simulink subsystem "Actuators"  (R2024b)
settings: Solver=VariableStepAuto  StartTime=0.0  StopTime=10.0  RelTol=1e-3
undefined symbols (not defined in the file): actuators, simulation
settings Model: Creator=marco  LastModifiedBy=domac

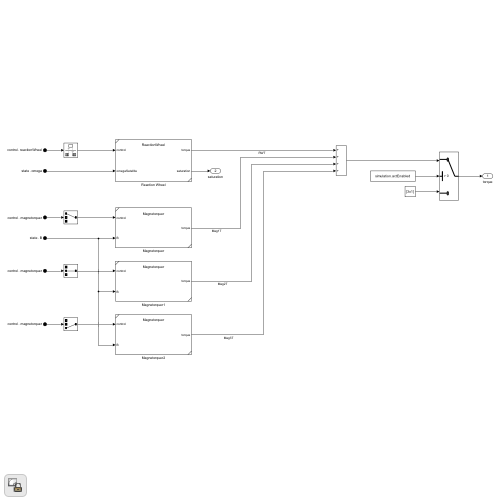
[thumbnail: Simulink's stored preview of the top-level diagram]
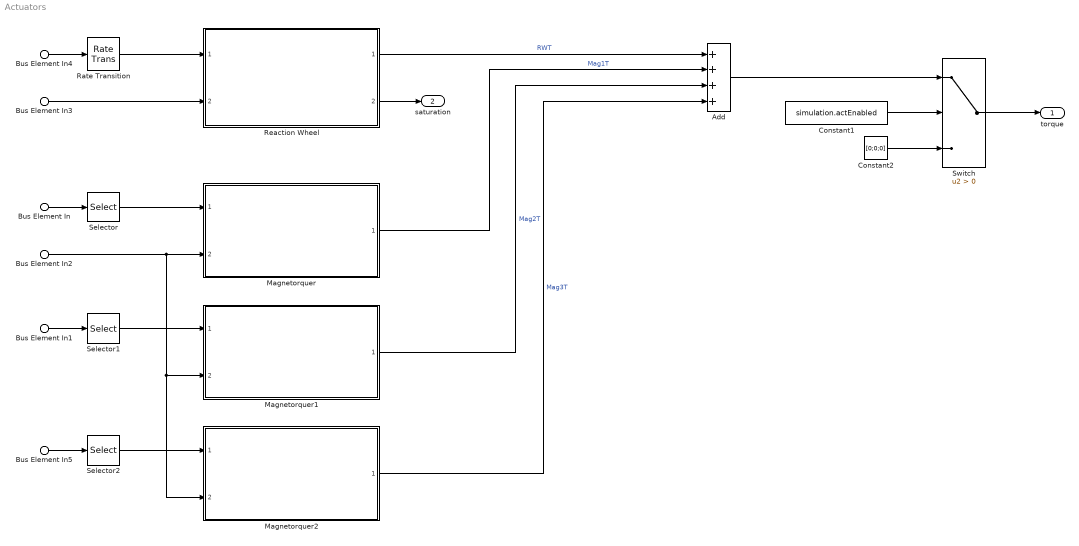
== system Actuators ==
  Bus Element In : Inport  PortName=control  Element=magnetorquer
  Bus Element In1 : Inport  PortName=control  Element=magnetorquer
  Bus Element In5 : Inport  PortName=control  Element=magnetorquer
  Bus Element In4 : Inport  PortName=control  Element=reactionWheel
  Bus Element In2 : Inport  Port=2  PortName=state  Element=B
  Bus Element In3 : Inport  Port=2  PortName=state  Element=omega
  Add : Sum  Inputs=++++
  Constant1 : Constant  Value=simulation.actEnabled
  Constant2 : Constant  Value=[0;0;0]  VectorParams1D=off
  Magnetorquer : Subsystem  ReferencedSubsystem=Magnetorquer  R=actuators.magnetorquer(1).R  k=actuators.magnetorquer(1).k
  Magnetorquer1 : Subsystem  ReferencedSubsystem=Magnetorquer  R=actuators.magnetorquer(2).R  k=actuators.magnetorquer(2).k
  Magnetorquer2 : Subsystem  ReferencedSubsystem=Magnetorquer  R=actuators.magnetorquer(3).R  k=actuators.magnetorquer(3).k
  Rate Transition : RateTransition  OutPortSampleTime=actuators.wheel.sTControl
  Reaction Wheel : Subsystem  ReferencedSubsystem=ReactionWheel  k=actuators.wheel.k  maxSpeed=actuators.wheel.maxSpeed  capacity=actuators.wheel.capacity  imbalance=actuators.wheel.imbalance  R=actuators.wheel.R  seed=0  torqueVariance=actuators.wheel.torqueVariance
  Selector : Selector  InputPortWidth=3  IndexOptions=Index vector (dialog)  Indices=1  OutputSizes=1
  Selector1 : Selector  InputPortWidth=3  IndexOptions=Index vector (dialog)  Indices=2  OutputSizes=1
  Selector2 : Selector  InputPortWidth=3  IndexOptions=Index vector (dialog)  Indices=3  OutputSizes=1
  Switch : Switch  Criteria=u2 > Threshold  SaturateOnIntegerOverflow=off  InputSameDT=off
  torque : Outport
  saturation : Outport  Port=2
  wires:
  Magnetorquer/1 -> Add/2  "Mag1T"
  Bus Element In2/1 -> Magnetorquer2/2, Magnetorquer1/2, Magnetorquer/2
  Bus Element In/1 -> Selector/1
  Selector/1 -> Magnetorquer/1
  Bus Element In4/1 -> Rate Transition/1
  Add/1 -> Switch/1
  Reaction Wheel/2 -> saturation/1
  Bus Element In1/1 -> Selector1/1
  Bus Element In5/1 -> Selector2/1
  Selector2/1 -> Magnetorquer2/1
  Selector1/1 -> Magnetorquer1/1
  Magnetorquer1/1 -> Add/3  "Mag2T"
  Magnetorquer2/1 -> Add/4  "Mag3T"
  Reaction Wheel/1 -> Add/1  "RWT"
  Constant1/1 -> Switch/2
  Constant2/1 -> Switch/3
  Switch/1 -> torque/1
  Bus Element In3/1 -> Reaction Wheel/2
  Rate Transition/1 -> Reaction Wheel/1
